simulink model "current_source_A_test"  (R2018b)
settings: Solver=VariableStepAuto  StartTime=0.0  StopTime=45  RelTol=1e-3
PreLoadFcn:
  | load_system('../simulink_reference_models/test_sequence_lib');
InitFcn:
  | close all
  | clear all
  | 
  | T_CNTL = 1/5e3;
  | 
  | VLL_NOM = 35e3;
  | F_NOM = 60;
libraries: simulink x22, test_sequence_lib x4
settings Model: SimulationMode=accelerator  Creator=HussamAlatrash  LastModifiedBy=ahhei
settings DataIOCC: ReturnWorkspaceOutputs=on
settings DebuggingCC: UnconnectedInputMsg=none  UnconnectedOutputMsg=none  UnconnectedLineMsg=none
settings ModelReferenceCC: EnableRefExpFcnMdlSchedulingChecks=off
settings RTWCC: Description=Generic Real-Time Target
settings ConfigComp: CovBoundaryAbsTol=1.0e-5

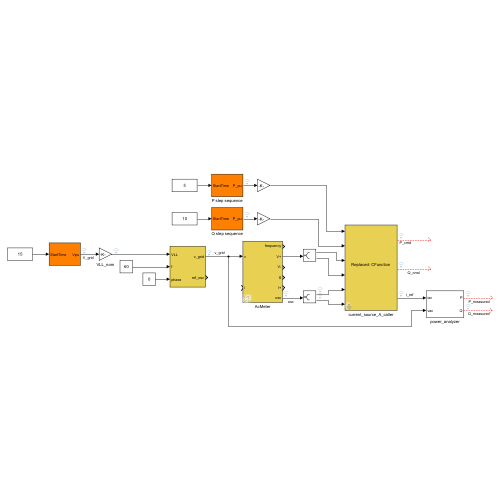
[thumbnail: Simulink's stored preview of the top-level diagram]
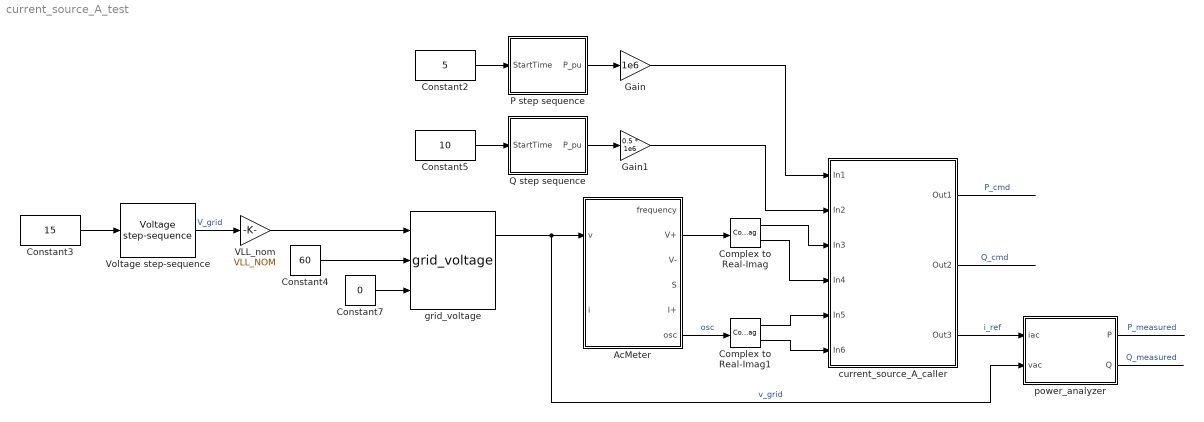
== system current_source_A_test ==
  AcMeter : Subsystem  AncestorBlock=test_sequence_lib/AcMeter
  Complex to Real-Imag : ComplexToRealImag
  Complex to Real-Imag1 : ComplexToRealImag
  Constant2 : Constant  Value=5
  Constant3 : Constant  Value=15
  Constant4 : Constant  Value=60
  Constant5 : Constant  Value=10
  Constant7 : Constant  Value=0
  Gain : Gain  Gain=1e6
  Gain1 : Gain  Gain=0.5 * 1e6
  P step sequence : Subsystem
  Q step sequence : Subsystem
  VLL_nom : Gain  Gain=VLL_NOM
  Voltage step-sequence : test_sequence_lib/Voltage step-sequence  SystemSampleTime=-1  EmptyChoice=off  PassThrough=off  PassThroughVariantControl=(default)  EmptyChoiceVariantControl=(default)  Latency=0  AutoFrameSizeCalculation=off
  current_source_A_caller : Subsystem  Description=Replaced Block  mask(Replaced Block){}
      mask help: This block has been replaced with an empty subsystem because it used functionality that is unavailable in Simulink R2018b.
      mask Display: fprintf('Replaced: %s\n','CFunction')
  grid_voltage : test_sequence_lib/grid_voltage  SystemSampleTime=-1  EmptyChoice=off  PassThrough=off  PassThroughVariantControl=(default)  EmptyChoiceVariantControl=(default)  Latency=0  AutoFrameSizeCalculation=off
  power_analyzer : Subsystem
  wires:
  Constant3/1 -> Voltage step-sequence/1
  grid_voltage/1 -> power_analyzer/2(vac), AcMeter/1(v)  "v_grid"
  VLL_nom/1 -> grid_voltage/1
  AcMeter/2(V+) -> Complex to Real-Imag/1
  Complex to Real-Imag/1 -> current_source_A_caller/3(In3)
  Complex to Real-Imag/2 -> current_source_A_caller/4(In4)
  Complex to Real-Imag1/1 -> current_source_A_caller/5(In5)
  Complex to Real-Imag1/2 -> current_source_A_caller/6(In6)
  AcMeter/6(osc) -> Complex to Real-Imag1/1  "osc"
  current_source_A_caller/3(Out3) -> power_analyzer/1(iac)  "i_ref"
  Gain/1 -> current_source_A_caller/1(In1)
  Gain1/1 -> current_source_A_caller/2(In2)
  Voltage step-sequence/1 -> VLL_nom/1  "V_grid"
  power_analyzer/1(P) -> ?  "P_measured"
  power_analyzer/2(Q) -> ?  "Q_measured"
  Constant7/1 -> grid_voltage/3
  Constant4/1 -> grid_voltage/2
  current_source_A_caller/2(Out2) -> ?  "Q_cmd"
  current_source_A_caller/1(Out1) -> ?  "P_cmd"
  Constant2/1 -> P step sequence/1(StartTime)
  Constant5/1 -> Q step sequence/1(StartTime)
  P step sequence/1(P_pu) -> Gain/1
  Q step sequence/1(P_pu) -> Gain1/1

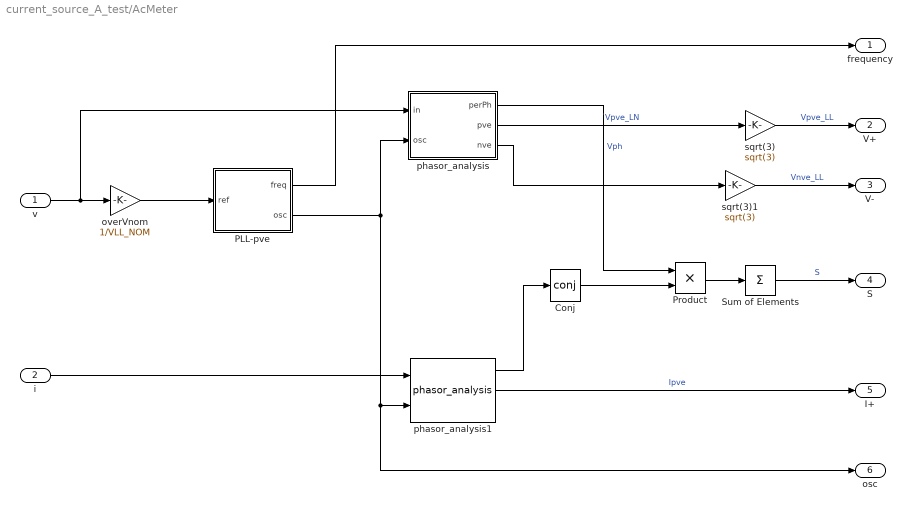
== system current_source_A_test/AcMeter ==
  v : Inport
  i : Inport  Port=2
  Conj : Math  Operator=conj  SaturateOnIntegerOverflow=on
  PLL-pve : Subsystem
  Product : Product
  Sum of Elements : Sum  Inputs=+
  overVnom : Gain  Gain=1/VLL_NOM
  phasor_analysis : Subsystem
  phasor_analysis1 : test_sequence_lib/AcMeter/phasor_analysis  SystemSampleTime=-1  EmptyChoice=off  PassThrough=off  PassThroughVariantControl=(default)  EmptyChoiceVariantControl=(default)  Latency=0  AutoFrameSizeCalculation=off
  sqrt(3) : Gain  Gain=sqrt(3)
  sqrt(3)1 : Gain  Gain=sqrt(3)
  frequency : Outport
  V+ : Outport  Port=2
  V- : Outport  Port=3
  S : Outport  Port=4
  I+ : Outport  Port=5
  osc : Outport  Port=6
  wires:
  PLL-pve/2(osc) -> phasor_analysis/2(osc), osc/1, phasor_analysis1/2
  phasor_analysis/1(perPh) -> Product/1  "Vph"
  Sum of Elements/1 -> S/1  "S"
  v/1 -> overVnom/1, phasor_analysis/1(in)
  PLL-pve/1(freq) -> frequency/1
  phasor_analysis1/1 -> Conj/1
  overVnom/1 -> PLL-pve/1(ref)
  Conj/1 -> Product/2
  Product/1 -> Sum of Elements/1
  phasor_analysis/2(pve) -> sqrt(3)/1  "Vpve_LN"
  phasor_analysis/3(nve) -> sqrt(3)1/1
  phasor_analysis1/2 -> I+/1  "Ipve"
  sqrt(3)1/1 -> V-/1  "Vnve_LL"
  i/1 -> phasor_analysis1/1
  sqrt(3)/1 -> V+/1  "Vpve_LL"

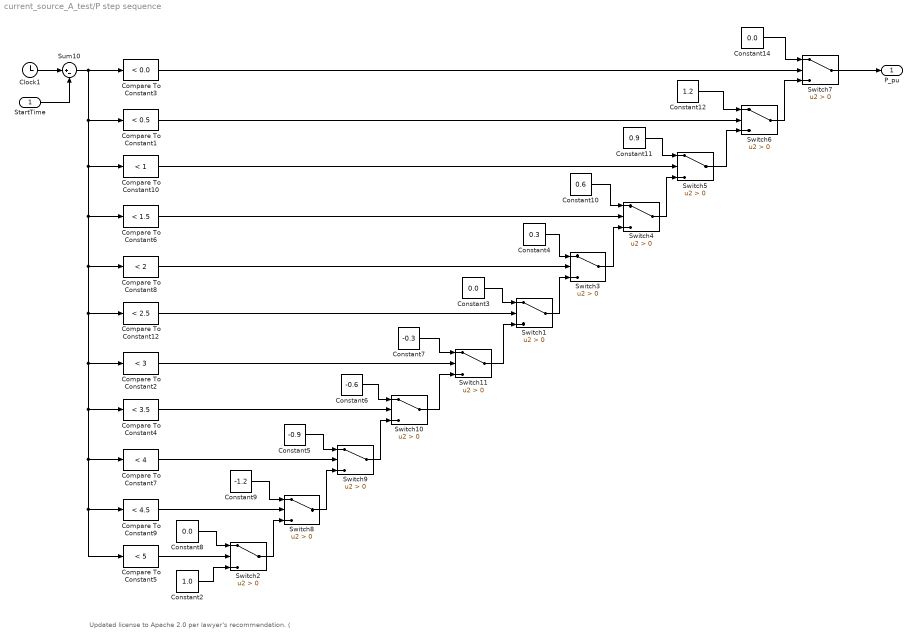
== system current_source_A_test/P step sequence ==
  note: Updated license to Apache 2.0 per lawyer's recommendation. (
  StartTime : Inport
  Clock1 : Clock
  Compare To Constant1 : simulink/Logic and Bit Operations/Compare To Constant  relop=<  const=0.5  OutDataTypeStr=boolean
  Compare To Constant10 : simulink/Logic and Bit Operations/Compare To Constant  relop=<  const=1  OutDataTypeStr=boolean
  Compare To Constant12 : simulink/Logic and Bit Operations/Compare To Constant  relop=<  const=2.5  OutDataTypeStr=boolean
  Compare To Constant2 : simulink/Logic and Bit Operations/Compare To Constant  relop=<  const=3  OutDataTypeStr=boolean
  Compare To Constant3 : simulink/Logic and Bit Operations/Compare To Constant  relop=<  const=0.0  OutDataTypeStr=boolean
  Compare To Constant4 : simulink/Logic and Bit Operations/Compare To Constant  relop=<  const=3.5  OutDataTypeStr=boolean
  Compare To Constant5 : simulink/Logic and Bit Operations/Compare To Constant  relop=<  const=5  OutDataTypeStr=boolean
  Compare To Constant6 : simulink/Logic and Bit Operations/Compare To Constant  relop=<  const=1.5  OutDataTypeStr=boolean
  Compare To Constant7 : simulink/Logic and Bit Operations/Compare To Constant  relop=<  const=4  OutDataTypeStr=boolean
  Compare To Constant8 : simulink/Logic and Bit Operations/Compare To Constant  relop=<  const=2  OutDataTypeStr=boolean
  Compare To Constant9 : simulink/Logic and Bit Operations/Compare To Constant  relop=<  const=4.5  OutDataTypeStr=boolean
  Constant10 : Constant  Value=0.6
  Constant11 : Constant  Value=0.9
  Constant12 : Constant  Value=1.2
  Constant14 : Constant  Value=0.0
  Constant2 : Constant  Value=1.0
  Constant3 : Constant  Value=0.0
  Constant4 : Constant  Value=0.3
  Constant5 : Constant  Value=-0.9
  Constant6 : Constant  Value=-0.6
  Constant7 : Constant  Value=-0.3
  Constant8 : Constant  Value=0.0
  Constant9 : Constant  Value=-1.2
  Sum10 : Sum  Inputs=|+-
  Switch{1..11} (11 alike) : Switch  Criteria=u2 > Threshold
  P_pu : Outport
  wires:
  StartTime/1 -> Sum10/2
  Clock1/1 -> Sum10/1
  Switch7/1 -> P_pu/1
  Switch6/1 -> Switch7/3
  Constant14/1 -> Switch7/1
  Compare To Constant3/1 -> Switch7/2
  Compare To Constant1/1 -> Switch6/2
  Constant12/1 -> Switch6/1
  Switch5/1 -> Switch6/3
  Switch4/1 -> Switch5/3
  Switch3/1 -> Switch4/3
  Switch1/1 -> Switch3/3
  Constant11/1 -> Switch5/1
  Constant10/1 -> Switch4/1
  Compare To Constant6/1 -> Switch4/2
  Compare To Constant8/1 -> Switch3/2
  Constant4/1 -> Switch3/1
  Compare To Constant10/1 -> Switch5/2
  Constant3/1 -> Switch1/1
  Compare To Constant12/1 -> Switch1/2
  Compare To Constant9/1 -> Switch8/2
  Compare To Constant7/1 -> Switch9/2
  Compare To Constant4/1 -> Switch10/2
  Compare To Constant5/1 -> Switch2/2
  Compare To Constant2/1 -> Switch11/2
  Switch9/1 -> Switch10/3
  Switch8/1 -> Switch9/3
  Constant2/1 -> Switch2/3
  Constant7/1 -> Switch11/1
  Constant9/1 -> Switch8/1
  Constant5/1 -> Switch9/1
  Constant8/1 -> Switch2/1
  Switch11/1 -> Switch1/3
  Constant6/1 -> Switch10/1
  Sum10/1 -> Compare To Constant3/1, Compare To Constant1/1, Compare To Constant10/1, Compare To Constant6/1, Compare To Constant8/1, Compare To Constant2/1, Compare To Constant4/1, Compare To Constant7/1, Compare To Constant5/1, Compare To Constant9/1, Compare To Constant12/1
  Switch2/1 -> Switch8/3
  Switch10/1 -> Switch11/3

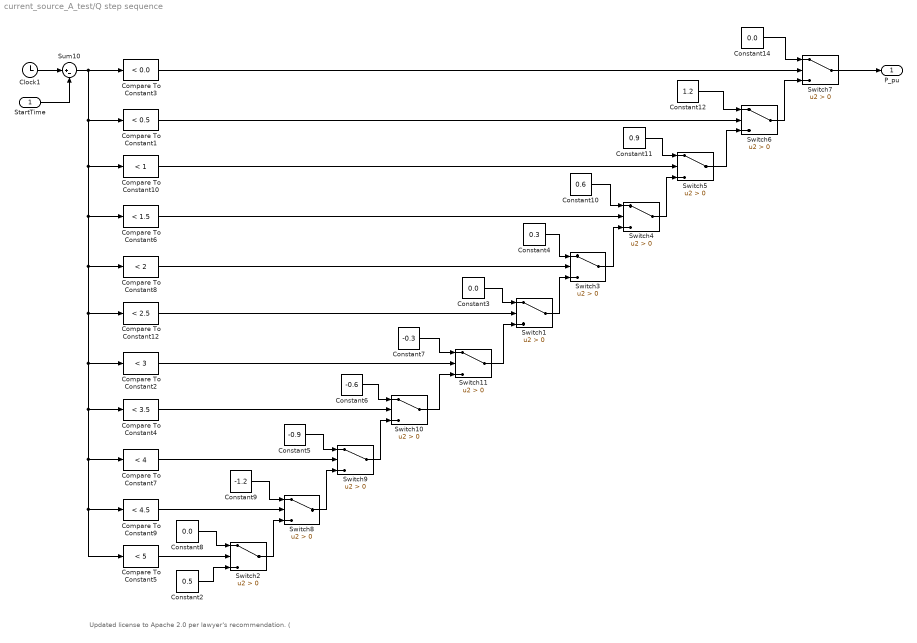
== system current_source_A_test/Q step sequence ==
  note: Updated license to Apache 2.0 per lawyer's recommendation. (
  StartTime : Inport
  Clock1 : Clock
  Compare To Constant1 : simulink/Logic and Bit Operations/Compare To Constant  relop=<  const=0.5  OutDataTypeStr=boolean
  Compare To Constant10 : simulink/Logic and Bit Operations/Compare To Constant  relop=<  const=1  OutDataTypeStr=boolean
  Compare To Constant12 : simulink/Logic and Bit Operations/Compare To Constant  relop=<  const=2.5  OutDataTypeStr=boolean
  Compare To Constant2 : simulink/Logic and Bit Operations/Compare To Constant  relop=<  const=3  OutDataTypeStr=boolean
  Compare To Constant3 : simulink/Logic and Bit Operations/Compare To Constant  relop=<  const=0.0  OutDataTypeStr=boolean
  Compare To Constant4 : simulink/Logic and Bit Operations/Compare To Constant  relop=<  const=3.5  OutDataTypeStr=boolean
  Compare To Constant5 : simulink/Logic and Bit Operations/Compare To Constant  relop=<  const=5  OutDataTypeStr=boolean
  Compare To Constant6 : simulink/Logic and Bit Operations/Compare To Constant  relop=<  const=1.5  OutDataTypeStr=boolean
  Compare To Constant7 : simulink/Logic and Bit Operations/Compare To Constant  relop=<  const=4  OutDataTypeStr=boolean
  Compare To Constant8 : simulink/Logic and Bit Operations/Compare To Constant  relop=<  const=2  OutDataTypeStr=boolean
  Compare To Constant9 : simulink/Logic and Bit Operations/Compare To Constant  relop=<  const=4.5  OutDataTypeStr=boolean
  Constant10 : Constant  Value=0.6
  Constant11 : Constant  Value=0.9
  Constant12 : Constant  Value=1.2
  Constant14 : Constant  Value=0.0
  Constant2 : Constant  Value=0.5
  Constant3 : Constant  Value=0.0
  Constant4 : Constant  Value=0.3
  Constant5 : Constant  Value=-0.9
  Constant6 : Constant  Value=-0.6
  Constant7 : Constant  Value=-0.3
  Constant8 : Constant  Value=0.0
  Constant9 : Constant  Value=-1.2
  Sum10 : Sum  Inputs=|+-
  Switch{1..11} (11 alike) : Switch  Criteria=u2 > Threshold
  P_pu : Outport
  wires:
  StartTime/1 -> Sum10/2
  Clock1/1 -> Sum10/1
  Switch7/1 -> P_pu/1
  Switch6/1 -> Switch7/3
  Constant14/1 -> Switch7/1
  Compare To Constant3/1 -> Switch7/2
  Compare To Constant1/1 -> Switch6/2
  Constant12/1 -> Switch6/1
  Switch5/1 -> Switch6/3
  Switch4/1 -> Switch5/3
  Switch3/1 -> Switch4/3
  Switch1/1 -> Switch3/3
  Constant11/1 -> Switch5/1
  Constant10/1 -> Switch4/1
  Compare To Constant6/1 -> Switch4/2
  Compare To Constant8/1 -> Switch3/2
  Constant4/1 -> Switch3/1
  Compare To Constant10/1 -> Switch5/2
  Constant3/1 -> Switch1/1
  Compare To Constant12/1 -> Switch1/2
  Compare To Constant9/1 -> Switch8/2
  Compare To Constant7/1 -> Switch9/2
  Compare To Constant4/1 -> Switch10/2
  Compare To Constant5/1 -> Switch2/2
  Compare To Constant2/1 -> Switch11/2
  Switch9/1 -> Switch10/3
  Switch8/1 -> Switch9/3
  Constant2/1 -> Switch2/3
  Constant7/1 -> Switch11/1
  Constant9/1 -> Switch8/1
  Constant5/1 -> Switch9/1
  Constant8/1 -> Switch2/1
  Switch11/1 -> Switch1/3
  Constant6/1 -> Switch10/1
  Sum10/1 -> Compare To Constant3/1, Compare To Constant1/1, Compare To Constant10/1, Compare To Constant6/1, Compare To Constant8/1, Compare To Constant2/1, Compare To Constant4/1, Compare To Constant7/1, Compare To Constant5/1, Compare To Constant9/1, Compare To Constant12/1
  Switch2/1 -> Switch8/3
  Switch10/1 -> Switch11/3

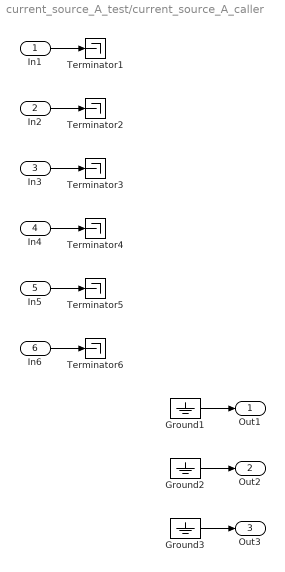
== system current_source_A_test/current_source_A_caller ==
  In1 : Inport
  In2 : Inport  Port=2
  In3 : Inport  Port=3
  In4 : Inport  Port=4
  In5 : Inport  Port=5
  In6 : Inport  Port=6
  Ground1 : Ground
  Ground2 : Ground
  Ground3 : Ground
  Terminator{1..6} (6 alike) : Terminator
  Out1 : Outport
  Out2 : Outport  Port=2
  Out3 : Outport  Port=3
  wires:
  Ground3/1 -> Out3/1
  Ground2/1 -> Out2/1
  Ground1/1 -> Out1/1
  In6/1 -> Terminator6/1
  In5/1 -> Terminator5/1
  In4/1 -> Terminator4/1
  In3/1 -> Terminator3/1
  In2/1 -> Terminator2/1
  In1/1 -> Terminator1/1

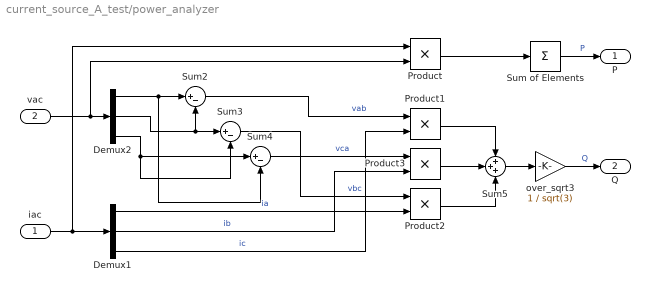
== system current_source_A_test/power_analyzer ==
  iac : Inport
  vac : Inport  Port=2
  Demux1 : Demux  Outputs=3
  Demux2 : Demux  Outputs=3
  Product{,1..3} (4 alike) : Product
  Sum of Elements : Sum  Inputs=+
  Sum2 : Sum  Inputs=|+-
  Sum3 : Sum  Inputs=|+-
  Sum4 : Sum  Inputs=|+-
  Sum5 : Sum  Inputs=+++
  over_sqrt3 : Gain  Gain=1 / sqrt(3)
  P : Outport
  Q : Outport  Port=2
  wires:
  Product/1 -> Sum of Elements/1
  Sum of Elements/1 -> P/1  "P"
  over_sqrt3/1 -> Q/1  "Q"
  Demux1/1 -> Product2/2  "ia"
  Demux2/1 -> Sum2/1, Sum4/2
  Sum2/1 -> Product1/1  "vab"
  Sum5/1 -> over_sqrt3/1
  Sum3/1 -> Product2/1  "vbc"
  iac/1 -> Product/1, Demux1/1
  vac/1 -> Product/2, Demux2/1
  Demux1/2 -> Product3/2  "ib"
  Demux1/3 -> Product1/2  "ic"
  Demux2/3 -> Sum3/2, Sum4/1
  Demux2/2 -> Sum2/2, Sum3/1
  Product3/1 -> Sum5/2
  Sum4/1 -> Product3/1  "vca"
  Product2/1 -> Sum5/3
  Product1/1 -> Sum5/1

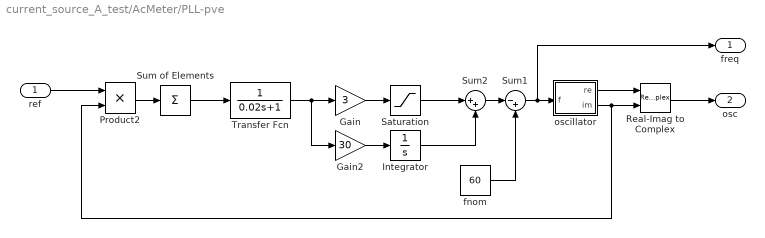
== system current_source_A_test/AcMeter/PLL-pve ==
  ref : Inport
  Gain : Gain  Gain=3
  Gain2 : Gain  Gain=30
  Integrator : Integrator  LimitOutput=on  UpperSaturationLimit=5  LowerSaturationLimit=-5
  Product2 : Product
  Real-Imag to Complex : RealImagToComplex
  Saturation : Saturate  UpperLimit=5  LowerLimit=-5
  Sum of Elements : Sum  Inputs=+
  Sum1 : Sum  Inputs=|-+
  Sum2 : Sum  Inputs=|++
  Transfer Fcn : TransferFcn  Denominator=[0.02 1]
  fnom : Constant  Value=60
  oscillator : Subsystem
  freq : Outport
  osc : Outport  Port=2
  wires:
  Gain2/1 -> Integrator/1
  Integrator/1 -> Sum2/2
  Sum2/1 -> Sum1/1
  fnom/1 -> Sum1/2
  Product2/1 -> Sum of Elements/1
  oscillator/2(im) -> Real-Imag to Complex/2, Product2/2
  Transfer Fcn/1 -> Gain/1, Gain2/1
  Saturation/1 -> Sum2/1
  Gain/1 -> Saturation/1
  Sum1/1 -> freq/1, oscillator/1(f)
  ref/1 -> Product2/1
  oscillator/1(re) -> Real-Imag to Complex/1
  Real-Imag to Complex/1 -> osc/1
  Sum of Elements/1 -> Transfer Fcn/1

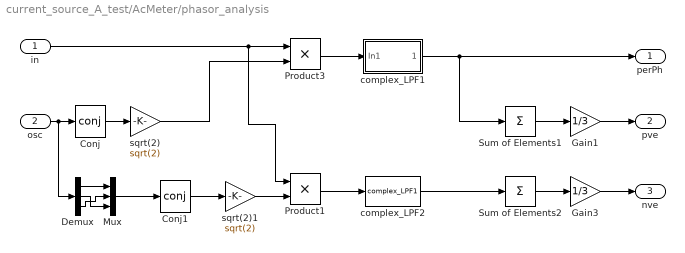
== system current_source_A_test/AcMeter/phasor_analysis ==
  in : Inport
  osc : Inport  Port=2
  Conj : Math  Operator=conj  SaturateOnIntegerOverflow=on
  Conj1 : Math  Operator=conj  SaturateOnIntegerOverflow=on
  Demux : Demux  Outputs=3
  Gain1 : Gain  Gain=1/3
  Gain3 : Gain  Gain=1/3
  Mux : Mux  Inputs=3
  Product1 : Product
  Product3 : Product
  Sum of Elements1 : Sum  Inputs=+
  Sum of Elements2 : Sum  Inputs=+
  complex_LPF1 : Subsystem  mask{wLPF=50}
      mask prompts: wLPF "Bandwidth (rad/sec)"
  complex_LPF2 : test_sequence_lib/AcMeter/phasor_analysis/complex_LPF1  wLPF=50
  sqrt(2) : Gain  Gain=sqrt(2)
  sqrt(2)1 : Gain  Gain=sqrt(2)
  perPh : Outport
  pve : Outport  Port=2
  nve : Outport  Port=3
  wires:
  complex_LPF2/1 -> Sum of Elements2/1
  Product1/1 -> complex_LPF2/1
  complex_LPF1/1(1) -> perPh/1, Sum of Elements1/1
  Product3/1 -> complex_LPF1/1(In1)
  Sum of Elements1/1 -> Gain1/1
  in/1 -> Product3/1, Product1/1
  osc/1 -> Demux/1, Conj/1
  Conj/1 -> sqrt(2)/1
  sqrt(2)/1 -> Product3/2
  Gain1/1 -> pve/1
  Demux/1 -> Mux/1
  Demux/2 -> Mux/3
  Demux/3 -> Mux/2
  Mux/1 -> Conj1/1
  Conj1/1 -> sqrt(2)1/1
  sqrt(2)1/1 -> Product1/2
  Sum of Elements2/1 -> Gain3/1
  Gain3/1 -> nve/1

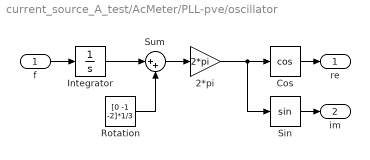
== system current_source_A_test/AcMeter/PLL-pve/oscillator ==
  f : Inport
  2*pi : Gain  Gain=2*pi
  Cos : Trigonometry  Operator=cos
  Integrator : Integrator
  Rotation : Constant  Value=[0 -1 -2]*1/3
  Sin : Trigonometry
  Sum : Sum  Inputs=|++
  re : Outport
  im : Outport  Port=2
  wires:
  2*pi/1 -> Sin/1, Cos/1
  f/1 -> Integrator/1
  Cos/1 -> re/1
  Sin/1 -> im/1
  Sum/1 -> 2*pi/1
  Integrator/1 -> Sum/1
  Rotation/1 -> Sum/2

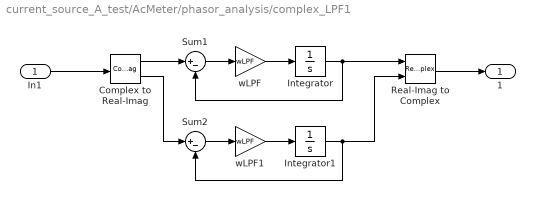
== system current_source_A_test/AcMeter/phasor_analysis/complex_LPF1 ==
  In1 : Inport
  Complex to Real-Imag : ComplexToRealImag
  Integrator : Integrator
  Integrator1 : Integrator
  Real-Imag to Complex : RealImagToComplex
  Sum1 : Sum  Inputs=|+-
  Sum2 : Sum  Inputs=|+-
  wLPF : Gain  Gain=wLPF
  wLPF1 : Gain  Gain=wLPF
  1 : Outport
  wires:
  Complex to Real-Imag/2 -> Sum2/1
  Sum2/1 -> wLPF1/1
  wLPF1/1 -> Integrator1/1
  Integrator1/1 -> Sum2/2, Real-Imag to Complex/2
  Real-Imag to Complex/1 -> 1/1
  In1/1 -> Complex to Real-Imag/1
  Integrator/1 -> Real-Imag to Complex/1, Sum1/2
  wLPF/1 -> Integrator/1
  Sum1/1 -> wLPF/1
  Complex to Real-Imag/1 -> Sum1/1
